simulink model "fir_blackbox"  (R2026a)
settings: Solver=FixedStepDiscrete  StopTime=300  FixedStep=1
model workspace (MAT data in the model file):
  b = [0.125 0.375 0.375 0.125]
  f_noise = 0.4
  f_sig = 0.01
libraries: simulink x1
settings Model: Creator=KoayXianCong  LastModifiedBy=KoayXianCong

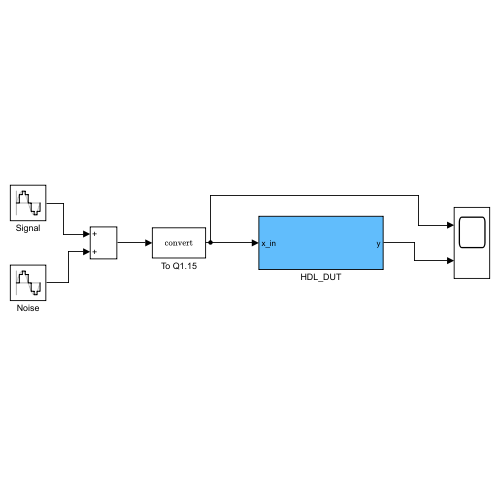
[thumbnail: Simulink's stored preview of the top-level diagram]
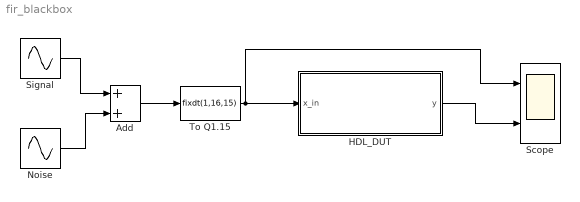
== system fir_blackbox ==
  Add : Sum
  HDL_DUT : Subsystem
  Noise : Sin  Amplitude=0.4  Frequency=2*pi*f_noise  SampleTime=1
  Scope : Scope  NumInputPorts=2
  Signal : Sin  Amplitude=0.5  Frequency=2*pi*f_sig  SampleTime=1
  To Q1.15 : DataTypeConversion  OutDataTypeStr=fixdt(1,16,15)  RndMeth=Nearest
  wires:
  Signal/1 -> Add/1
  Noise/1 -> Add/2
  Add/1 -> To Q1.15/1
  To Q1.15/1 -> HDL_DUT/1(x_in), Scope/1
  HDL_DUT/1(y) -> Scope/2

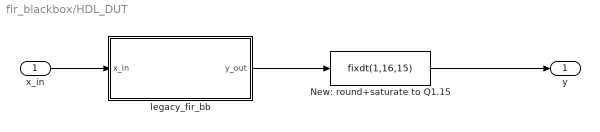
== system fir_blackbox/HDL_DUT ==
  x_in : Inport
  New: round+saturate to Q1.15 : DataTypeConversion  OutDataTypeStr=fixdt(1,16,15)  RndMeth=Nearest
  legacy_fir_bb : Subsystem
  y : Outport
  wires:
  x_in/1 -> legacy_fir_bb/1(x_in)
  legacy_fir_bb/1(y_out) -> New: round+saturate to Q1.15/1
  New: round+saturate to Q1.15/1 -> y/1

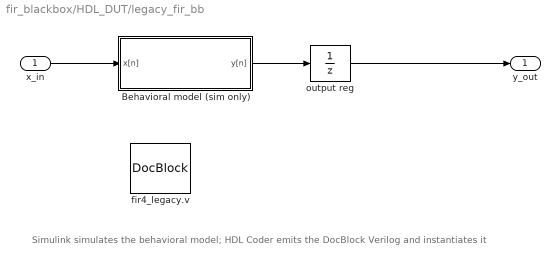
== system fir_blackbox/HDL_DUT/legacy_fir_bb ==
  note: Simulink simulates the behavioral model; HDL Coder emits the DocBlock Verilog and instantiates it
  x_in : Inport
  Behavioral model (sim only) : Subsystem
  fir4_legacy.v : simulink/Model-Wide Utilities/DocBlock  DocumentType=Text
      content=|
      | // -----------------------------------------------------------------------------
      | // fir4_legacy.v
      | // "Legacy" hand-written RTL used in Part 2 (HDL import) and Part 4 (cosimulation)
      | //
      | // 4-tap low-pass FIR:  y[n] = ( x[n] + 3*x[n-1] + 3*x[n-2] + x[n-3] ) / 8
      | //
      | //   x_in  : signed 16-bit, Q1.15  (Simulink: fixdt(1,16,15))
      | //   y_out : signed 19-bit, Q4.18  (Simulink: fixdt(1,19,18))  -- full precision, no rounding
      | //   Latency: 1 clock (registered output)
      | // -----------------------------------------------------------------------------
      | module fir4_legacy (
      |     input  wire               clk,
      |     input  wire               rst,      // synchronous, active-high
      |     input  wire               clk_en,
      |     input  wire signed [15:0] x_in,
      |     output reg  signed [18:0] y_out
      | );
      |
      |     // tapped delay line
      |     reg signed [15:0] x_d1;
      |     reg signed [15:0] x_d2;
      |     reg signed [15:0] x_d3;
      |
      |     // coefficients 1,3,3,1 (the /8 is a binary-point shift: Q1.15 -> Q4.18)
      |     wire signed [18:0] tap0 = x_in;
      |     wire signed [18:0] tap1 = (x_d1 <<< 1) + x_d1;   // 3*x[n-1]
      |     wire signed [18:0] tap2 = (x_d2 <<< 1) + x_d2;   // 3*x[n-2]
      |     wire signed [18:0] tap3 = x_d3;
      |     wire signed [18:0] acc  = tap0 + tap1 + tap2 + tap3;
      |
      |     always @(posedge clk) begin
      |         if (rst) begin
      |             x_d1  <= 16'sd0;
      |             x_d2  <= 16'sd0;
      |             x_d3  <= 16'sd0;
      |             y_out <= 19'sd0;
      |         end else if (clk_en) begin
      |             x_d1  <= x_in;
      |             x_d2  <= x_d1;
      |             x_d3  <= x_d2;
      |             y_out <= acc;
      |         end
      |     end
      |
      | endmodule
  output reg : UnitDelay  SampleTime=-1
  y_out : Outport
  wires:
  x_in/1 -> Behavioral model (sim only)/1(x[n])
  Behavioral model (sim only)/1(y[n]) -> output reg/1
  output reg/1 -> y_out/1

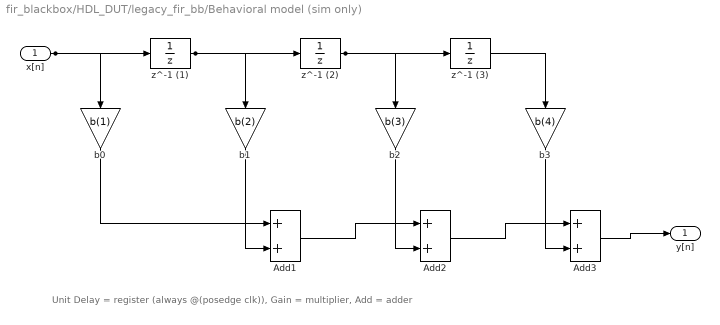
== system fir_blackbox/HDL_DUT/legacy_fir_bb/Behavioral model (sim only) ==
  note: Unit Delay = register (always @(posedge clk)), Gain = multiplier, Add = adder
  x[n] : Inport
  Add1 : Sum  OutDataTypeStr=fixdt(1,19,18)
  Add2 : Sum  OutDataTypeStr=fixdt(1,19,18)
  Add3 : Sum  OutDataTypeStr=fixdt(1,19,18)
  b0 : Gain  Gain=b(1)  ParamDataTypeStr=fixdt(1,16,15)  OutDataTypeStr=fixdt(1,19,18)
  b1 : Gain  Gain=b(2)  ParamDataTypeStr=fixdt(1,16,15)  OutDataTypeStr=fixdt(1,19,18)
  b2 : Gain  Gain=b(3)  ParamDataTypeStr=fixdt(1,16,15)  OutDataTypeStr=fixdt(1,19,18)
  b3 : Gain  Gain=b(4)  ParamDataTypeStr=fixdt(1,16,15)  OutDataTypeStr=fixdt(1,19,18)
  z^-1 (1) : UnitDelay  SampleTime=-1
  z^-1 (2) : UnitDelay  SampleTime=-1
  z^-1 (3) : UnitDelay  SampleTime=-1
  y[n] : Outport
  wires:
  Add3/1 -> y[n]/1
  b3/1 -> Add3/2
  Add2/1 -> Add3/1
  b2/1 -> Add2/2
  Add1/1 -> Add2/1
  b1/1 -> Add1/2
  b0/1 -> Add1/1
  z^-1 (3)/1 -> b3/1
  z^-1 (2)/1 -> b2/1, z^-1 (3)/1
  z^-1 (1)/1 -> b1/1, z^-1 (2)/1
  x[n]/1 -> b0/1, z^-1 (1)/1
